simulink model "Pack_Thermal"  (R2026b)
settings: Solver=VariableStepAuto
undefined symbols (not defined in the file or in its folder): P, Ts
libraries: fl_lib x14, nesl_utility x6
settings Model: Creator=aomar  LastModifiedBy=aomar

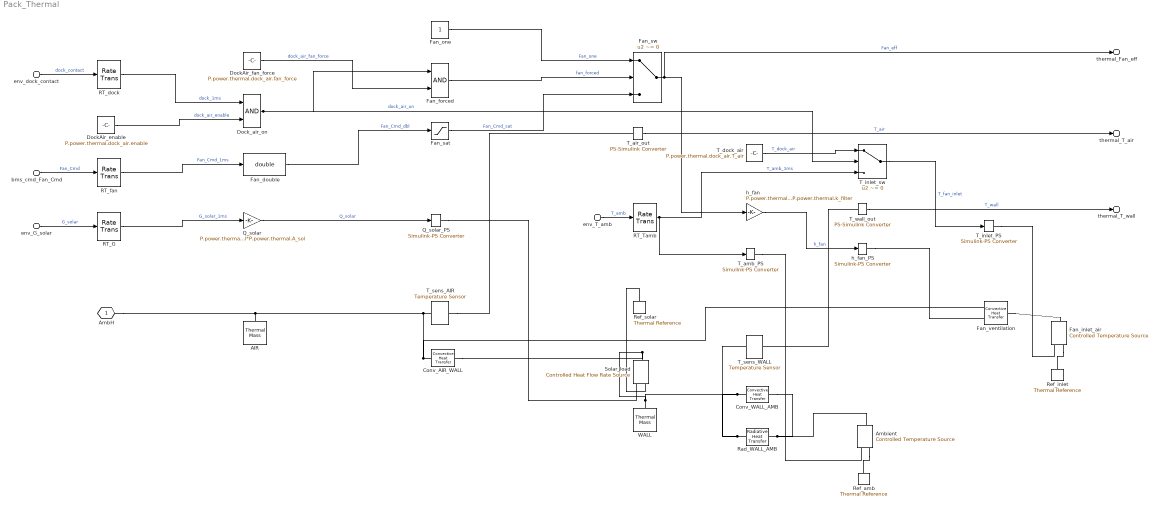
== system Pack_Thermal ==
  bms_cmd_Fan_Cmd : Inport  PortName=bms_cmd  Element=Fan_Cmd
  env_T_amb : Inport  Port=2  PortName=env  Element=T_amb
  env_G_solar : Inport  Port=2  PortName=env  Element=G_solar
  env_dock_contact : Inport  Port=2  PortName=env  Element=dock_contact
  AIR : fl_lib/Thermal/Thermal Elements/Thermal Mass  mass_type=foundation.enum.constant_variable.constant  mass=P.power.thermal.m_int kg  sp_heat=P.power.thermal.cp_int J/(K*kg)  mass_min=1e-6 kg  num_ports=foundation.enum.numPorts2.one  m_specify=off  m_priority=High  m=1 kg  m_nominal_specify=off  m_nominal_value=1  m_nominal_unit=kg  T_specify=on  T_priority=High  T=P.power.thermal.T_init_K K  T_nominal_specify=off  T_nominal_value=1  T_nominal_unit=K  Q_specify=off  Q_priority=None  Q=0 W  Q_nominal_specify=off  Q_nominal_value=1  Q_nominal_unit=W
  Ambient : fl_lib/Thermal/Thermal Sources/Controlled Temperature Source
  Conv_AIR_WALL : fl_lib/Thermal/Thermal Elements/Convective Heat Transfer  thermal_type=foundation.enum.constant_variable.constant  area=P.power.thermal.A_int m^2  heat_tr_coeff=P.power.thermal.h_in W/(K*m^2)  min_heat_tr_coeff=1e-3 W/(K*m^2)  T_specify=off  T_priority=None  T=0 K  T_nominal_specify=off  T_nominal_value=1  T_nominal_unit=K  Q_specify=off  Q_priority=None  Q=0 W  Q_nominal_specify=off  Q_nominal_value=1  Q_nominal_unit=W
  Conv_WALL_AMB : fl_lib/Thermal/Thermal Elements/Convective Heat Transfer  thermal_type=foundation.enum.constant_variable.constant  area=P.power.thermal.A_ext m^2  heat_tr_coeff=P.power.thermal.h_ext W/(K*m^2)  min_heat_tr_coeff=1e-3 W/(K*m^2)  T_specify=off  T_priority=None  T=0 K  T_nominal_specify=off  T_nominal_value=1  T_nominal_unit=K  Q_specify=off  Q_priority=None  Q=0 W  Q_nominal_specify=off  Q_nominal_value=1  Q_nominal_unit=W
  DockAir_enable : Constant  Value=P.power.thermal.dock_air.enable  OutDataTypeStr=boolean  SampleTime=Ts.base
  DockAir_fan_force : Constant  Value=P.power.thermal.dock_air.fan_force  OutDataTypeStr=boolean  SampleTime=Ts.base
  Dock_air_on : Logic  AllPortsSameDT=off  OutDataTypeStr=boolean
  Fan_double : DataTypeConversion  OutDataTypeStr=double  SaturateOnIntegerOverflow=off  RndMeth=Floor
  Fan_forced : Logic  AllPortsSameDT=off  OutDataTypeStr=boolean
  Fan_inlet_air : fl_lib/Thermal/Thermal Sources/Controlled Temperature Source
  Fan_one : Constant  SampleTime=Ts.base
  Fan_sat : Saturate  UpperLimit=1  LowerLimit=0
  Fan_sw : Switch  Criteria=u2 ~= 0  SaturateOnIntegerOverflow=off  InputSameDT=off
  Fan_ventilation : fl_lib/Thermal/Thermal Elements/Convective Heat Transfer  thermal_type=foundation.enum.constant_variable.variable  area=P.power.thermal.A_int m^2  heat_tr_coeff=20 W/(K*m^2)  min_heat_tr_coeff=1e-3 W/(K*m^2)  T_specify=off  T_priority=None  T=0 K  T_nominal_specify=off  T_nominal_value=1  T_nominal_unit=K  Q_specify=off  Q_priority=None  Q=0 W  Q_nominal_specify=off  Q_nominal_value=1  Q_nominal_unit=W
  Q_solar : Gain  Gain=P.power.thermal.alpha_sol*P.power.thermal.A_sol
  Q_solar_PS : nesl_utility/Simulink-PS Converter  PhysicalDomain=network_engine_domain  SubClassName=ps_input  LeftPortType=input  RightPortType=output  PseudoPeriodic=off  Frequencies=[]  NoiseDistribution=none  NoiseParameters=[]  Unit=W  AffineConversion=off  FilteringAndDerivatives=zero  SimscapeFilterOrder=1  InputFilterTimeConstant=0.001  UdotUserProvided=0
  RT_G : RateTransition  OutPortSampleTime=Ts.base
  RT_Tamb : RateTransition  OutPortSampleTime=Ts.base
  RT_dock : RateTransition  OutPortSampleTime=Ts.base
  RT_fan : RateTransition  OutPortSampleTime=Ts.base
  Rad_WALL_AMB : fl_lib/Thermal/Thermal Elements/Radiative Heat Transfer  area=P.power.thermal.A_ext m^2  rad_tr_coeff=P.power.thermal.rad_tr_coeff W/(K^4*m^2)  T_specify=off  T_priority=None  T=0 K  T_nominal_specify=off  T_nominal_value=1  T_nominal_unit=K  Q_specify=off  Q_priority=None  Q=0 W  Q_nominal_specify=off  Q_nominal_value=1  Q_nominal_unit=W
  Ref_amb : fl_lib/Thermal/Thermal Elements/Thermal Reference
  Ref_inlet : fl_lib/Thermal/Thermal Elements/Thermal Reference
  Ref_solar : fl_lib/Thermal/Thermal Elements/Thermal Reference
  Solar_load : fl_lib/Thermal/Thermal Sources/Controlled Heat Flow Rate Source
  T_air_out : nesl_utility/PS-Simulink Converter  PhysicalDomain=network_engine_domain  SubClassName=ps_output  LeftPortType=input  RightPortType=output  PseudoPeriodic=off  Frequencies=[]  VectorFormat=inherit  Unit=K  AffineConversion=off
  T_amb_PS : nesl_utility/Simulink-PS Converter  PhysicalDomain=network_engine_domain  SubClassName=ps_input  LeftPortType=input  RightPortType=output  PseudoPeriodic=off  Frequencies=[]  NoiseDistribution=none  NoiseParameters=[]  Unit=K  AffineConversion=off  FilteringAndDerivatives=zero  SimscapeFilterOrder=1  InputFilterTimeConstant=0.001  UdotUserProvided=0
  T_dock_air : Constant  Value=P.power.thermal.dock_air.T_air  SampleTime=Ts.base
  T_inlet_PS : nesl_utility/Simulink-PS Converter  PhysicalDomain=network_engine_domain  SubClassName=ps_input  LeftPortType=input  RightPortType=output  PseudoPeriodic=off  Frequencies=[]  NoiseDistribution=none  NoiseParameters=[]  Unit=K  AffineConversion=off  FilteringAndDerivatives=zero  SimscapeFilterOrder=1  InputFilterTimeConstant=0.001  UdotUserProvided=0
  T_inlet_sw : Switch  Criteria=u2 ~= 0  SaturateOnIntegerOverflow=off  InputSameDT=off
  T_sens_AIR : fl_lib/Thermal/Thermal Sensors/Temperature Sensor  temperature_measure=foundation.enum.MeasurementReference.absolute
  T_sens_WALL : fl_lib/Thermal/Thermal Sensors/Temperature Sensor  temperature_measure=foundation.enum.MeasurementReference.absolute
  T_wall_out : nesl_utility/PS-Simulink Converter  PhysicalDomain=network_engine_domain  SubClassName=ps_output  LeftPortType=input  RightPortType=output  PseudoPeriodic=off  Frequencies=[]  VectorFormat=inherit  Unit=K  AffineConversion=off
  WALL : fl_lib/Thermal/Thermal Elements/Thermal Mass  mass_type=foundation.enum.constant_variable.constant  mass=P.power.thermal.m_wall kg  sp_heat=P.power.thermal.cp_wall J/(K*kg)  mass_min=1e-6 kg  num_ports=foundation.enum.numPorts2.one  m_specify=off  m_priority=High  m=1 kg  m_nominal_specify=off  m_nominal_value=1  m_nominal_unit=kg  T_specify=on  T_priority=High  T=P.power.thermal.T_init_K K  T_nominal_specify=off  T_nominal_value=1  T_nominal_unit=K  Q_specify=off  Q_priority=None  Q=0 W  Q_nominal_specify=off  Q_nominal_value=1  Q_nominal_unit=W
  h_fan : Gain  Gain=P.power.thermal.h_fan*P.power.thermal.k_filter
  h_fan_PS : nesl_utility/Simulink-PS Converter  PhysicalDomain=network_engine_domain  SubClassName=ps_input  LeftPortType=input  RightPortType=output  PseudoPeriodic=off  Frequencies=[]  NoiseDistribution=none  NoiseParameters=[]  Unit=W/(m^2*K)  AffineConversion=off  FilteringAndDerivatives=zero  SimscapeFilterOrder=1  InputFilterTimeConstant=0.001  UdotUserProvided=0
  AmbH : PMIOPort  Side=Left  ConnectionType=Connection: foundation.thermal.thermal
  thermal_T_air : Outport  PortName=thermal  Element=T_air
  thermal_T_wall : Outport  PortName=thermal  Element=T_wall
  thermal_Fan_eff : Outport  PortName=thermal  Element=Fan_eff
  wires:
  env_dock_contact/1 -> RT_dock/1  "dock_contact"
  bms_cmd_Fan_Cmd/1 -> RT_fan/1  "Fan_Cmd"
  env_G_solar/1 -> RT_G/1  "G_solar"
  DockAir_enable/1 -> Dock_air_on/2  "dock_air_enable"
  RT_dock/1 -> Dock_air_on/1  "dock_1ms"
  RT_fan/1 -> Fan_double/1  "Fan_Cmd_1ms"
  RT_G/1 -> Q_solar/1  "G_solar_1ms"
  DockAir_fan_force/1 -> Fan_forced/2  "dock_air_fan_force"
  Dock_air_on/1 -> T_inlet_sw/2, Fan_forced/1  "dock_air_on"
  Q_solar/1 -> Q_solar_PS/1  "Q_solar"
  Fan_double/1 -> Fan_sat/1  "Fan_Cmd_dbl"
  Fan_one/1 -> Fan_sw/1  "Fan_one"
  Fan_forced/1 -> Fan_sw/2  "fan_forced"
  Fan_sat/1 -> Fan_sw/3  "Fan_Cmd_sat"
  env_T_amb/1 -> RT_Tamb/1  "T_amb"
  T_air_out/1 -> thermal_T_air/1  "T_air"
  RT_Tamb/1 -> T_inlet_sw/3, T_amb_PS/1  "T_amb_1ms"
  Fan_sw/1 -> h_fan/1, thermal_Fan_eff/1  "Fan_eff"
  T_dock_air/1 -> T_inlet_sw/1  "T_dock_air"
  h_fan/1 -> h_fan_PS/1  "h_fan"
  T_wall_out/1 -> thermal_T_wall/1  "T_wall"
  T_inlet_sw/1 -> T_inlet_PS/1  "T_fan_inlet"
  connections:
  AIR/LConn1 -- AmbH/RConn1 -- T_sens_AIR/LConn1 -- Conv_AIR_WALL/LConn1 -- Fan_ventilation/LConn1
  Rad_WALL_AMB/RConn1 -- Conv_WALL_AMB/RConn1 -- Ambient/LConn1
  T_amb_PS/RConn1 -- Ambient/RConn1
  Ambient/RConn2 -- Ref_amb/LConn1
  Solar_load/LConn1 -- Conv_AIR_WALL/RConn1 -- WALL/LConn1 -- Conv_WALL_AMB/LConn1 -- Rad_WALL_AMB/LConn1 -- T_sens_WALL/LConn1
  Fan_ventilation/RConn1 -- Fan_inlet_air/LConn1
  T_inlet_PS/RConn1 -- Fan_inlet_air/RConn1
  Fan_inlet_air/RConn2 -- Ref_inlet/LConn1
  h_fan_PS/RConn1 -- Fan_ventilation/LConn2
  Q_solar_PS/RConn1 -- Solar_load/RConn1
  Ref_solar/LConn1 -- Solar_load/RConn2
  T_sens_AIR/RConn1 -- T_air_out/LConn1
  T_wall_out/LConn1 -- T_sens_WALL/RConn1
